simulink model "ADCS_pointing_test"  (R2025b)
settings: Solver=VariableStepAuto  StartTime=0.0  StopTime=t0  FixedStep=0.1  MaxStep=0.1  RelTol=1e-3
values from neighbouring files (symbols this model uses):
  h0 = [1 1 1]*0.5    [parameters.m]
  kd_point = 20    [parameters.m]
  kp_point = 2    [parameters.m]
  omega_0 = [0 0 0.0011]    [parameters.m]
  P = satellite_params()    [individual_test_with_dynamics.m]    (also in parameters.m; test.m = thrusters(:, 1:3))
  q0 = [sqrt(0.5) -sqrt(0.5) 0 0]    [parameters.m]
  ts = 0.1    [parameters.m]
libraries: matrix_library x3, sim3dlib x2, aerolibutil x2
settings Model: Creator=ADMIN  LastModifiedBy=ADMIN
settings DataIOCC: ExternalInput=ds  LoadExternalInput=on

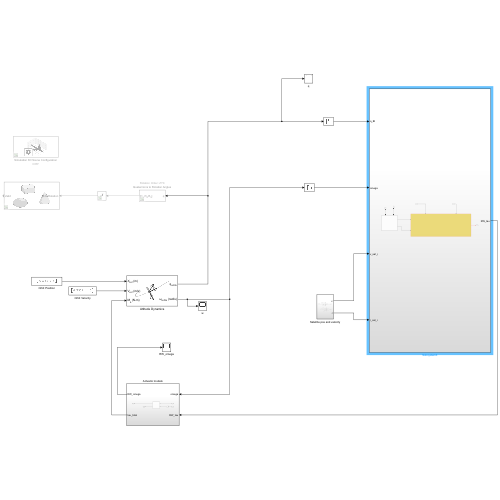
[thumbnail: Simulink's stored preview of the top-level diagram]
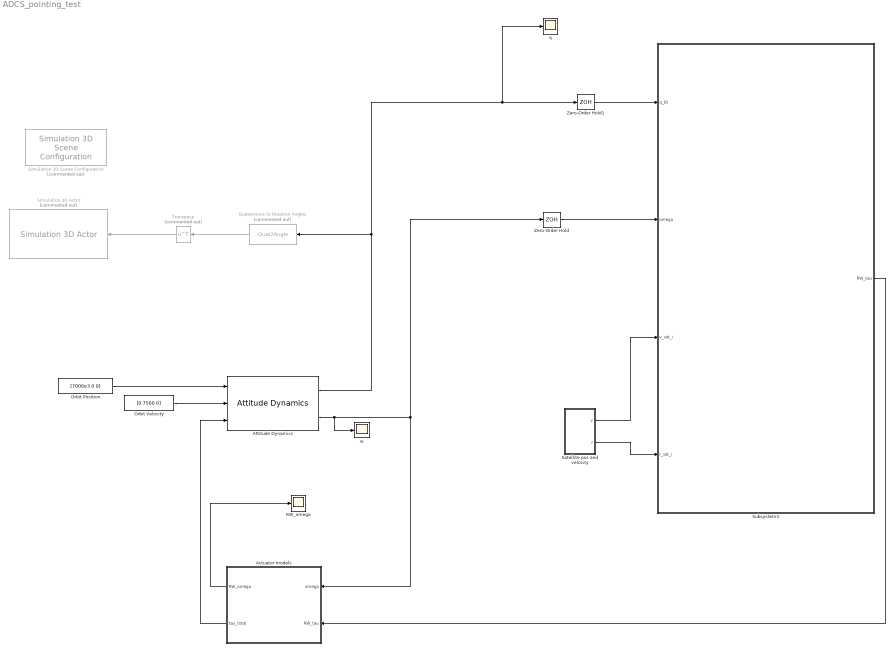
== system ADCS_pointing_test ==
  Actuator models : Subsystem
  Attitude Dynamics : AttitudeDynamics  dateOut=off  mass=P.mass0  inertia=P.I0  outputFuelStatus=off  attitude=q0.'  attitudeRate=omega_0.'  useGravGrad=off  angleUnits=Radians
  Orbit Position : Constant  Value=[7000e3 0 0]
  Orbit Velocity : Constant  Value=[0 7500 0]
  Quaternions to Rotation Angles : Quat2Angle  Commented=on
      settings: AttributesFormatString=Rotation Order: %<rotationOrder>
  RW_omega : Scope
      settings: ActiveDisplayYMinimum=-1.8375  ActiveDisplayYMaximum=1.8375  DataLoggingVariableName=ScopeData5
  Satellite pos and velocity : Subsystem
  Simulation 3D Actor : sim3dlib/Simulation 3D Actor  Priority=1  Commented=on  ActorName=M4V  ParentName=Scene Origin  Operation=Create at setup  InitScriptText=|  SampleTime=-1  Translation=[0 0 0]  Rotation=[0 0 0]  Scale=[1 1 1]*0.1  InputsText=M4V.Rotation  aMode=5  ActorTag=M4V  ActorType=Sim3dActor  ID=C
      | % Reserved keywords:
      | % - Actor : handle to this actor object
      | % - World : handle to the world object
      | 
      | % Examples:
      | 
      | % Create a primitive geometry (optional)
      | % createShape(Actor, 'box', [1 1 1]);
      | 
      | % Initialize values (optional)
      | % Actor.Physics = true;
      | % Actor.Color = [1 0 0];
      | M4V.Mobility = sim3d.utils.MobilityTypes.Movable;
      | 
      | % For simple motion without gravity
      | M4V.Physics = true;
      | M4V.Gravity = false;
      | M4V.Collisions = false;
  Simulation 3D Scene Configuration : sim3dlib/Simulation 3D Scene Configuration  Priority=0  Commented=on  ProjectFormat=Default Scenes  SceneDesc=Space  ProjectName=C:\Program Files\MATLAB\R2025b\toolbox\shared\sim3d_projects\automotive_project_windows\UE\WindowsNoEditor\VehicleSimulation.exe  ScenePath=/Game/Maps/HwStrght  EnableOpenDRIVE=off  vehTagList={'Custom';'M4V';'Scene Origin'}  vehTag=Custom  AttachedCameraRelativeTranslation=[-20000 0 0]  FreeCameraDefaultInitialTranslation=[-6, 0, 2]  AttachedCameraRelativeRotation=[0 0 0]  FreeCameraDefaultInitialRotation=[0, -15, 0]  ViewpointName=Custom  FreeCameraInitialTranslation=[-1500 0 500]  ViewpointTranslation=[0 0 0]  FreeCameraInitialRotation=[0 0 0]  ViewpointRotation=[0 0 0]  OpVisEn=off  Ts=1  EnableWindow=on  EnableRemoteAccess=off  EnableWeather=off  SunAzimuth=90  SunAltitude=40.0  EnableGeospatialSun=off  Latitude=0  Longitude=0  Date=2023-01-01  Time=10:30:00  GeoTimeZone=-5.0  SunDaylightSaving=off  wind=0  clouds=10  EnableVolumetricClouds=off  CloudCoverage=0  CloudAltitude=6  fog=0  rain=0  RaindropsEffect=off  SnowDensity=0  EnableGeospatial=off  TilesetSource=Earth terrain  UseTrueOrigin=off  OriginHeight=200  OriginLatitude=40.744652  OriginLongitude=-73.988864  MapStyle=Aerial  AdditionalAssetIDs=[]  UseAdvancedSunSky=off  SolarTime=11  TimeZone=-5  Day=21  Month=9  Year=2022  UseDaylightSavingTime=on  DSTStartDay=10  DSTStartMonth=3  DSTEndDay=3  DSTEndMonth=11  DSTSwitchHour=2  sensorTag=MainCamera1  sensorId=1  sensorName=MainCamera1  mountLoc=Origin  offsetFlag=off  tmountOffset=[0, 0, 0]  rmountOffset=[0, 0, 0]  HorizontalResolution=1280  VerticalResolution=720  HorizontalFOV=60  mountPoint=[0 0 0]  mountOrientation=[0 0 0]  aMode=0  ID=1  GeoTrigger=Inactive  ViewNameList={'Custom'}  ViewTranslationList={'[-1500 0 500]'}  ViewRotationList={'[0 0 0]'}
      settings: AttributesFormatString=ICRF  LibrarySourceBlock=aerolibsim3d/Simulation 3D Scene Configuration
  Subsystem3 : Subsystem
  Transpose : Math  Commented=on  Operator=transpose
  Zero-Order Hold : ZeroOrderHold  SampleTime=ts
  Zero-Order Hold1 : ZeroOrderHold  SampleTime=ts
  q : Scope
      settings: ActiveDisplayYMinimum=-1.2475163124751956  ActiveDisplayYMaximum=1.2496817270129896  DataLoggingVariableName=ScopeData2
  w : Scope
      settings: ActiveDisplayYMinimum=-0.031776762100484128  ActiveDisplayYMaximum=0.0395431946397378
  wires:
  Orbit Position/1 -> Attitude Dynamics/1
  Orbit Velocity/1 -> Attitude Dynamics/2
  Subsystem3/1(RW_tau) -> Actuator models/2(RW_tau)
  Actuator models/2(tau_total) -> Attitude Dynamics/3
  Transpose/1 -> Simulation 3D Actor/1
  Quaternions to Rotation Angles/1 -> Transpose/1
  Attitude Dynamics/2 -> w/1, Zero-Order Hold/1, Actuator models/1(omega)
  Actuator models/1(RW_omega) -> RW_omega/1
  Satellite pos and velocity/1(v) -> Subsystem3/3(v_sat_i)
  Satellite pos and velocity/2(r) -> Subsystem3/4(r_sat_i)
  Zero-Order Hold/1 -> Subsystem3/2(omega)
  Zero-Order Hold1/1 -> Subsystem3/1(q_BI)
  Attitude Dynamics/1 -> q/1, Zero-Order Hold1/1, Quaternions to Rotation Angles/1

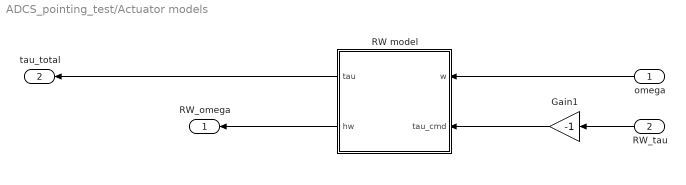
== system ADCS_pointing_test/Actuator models ==
  omega : Inport
  RW_tau : Inport  Port=2
  Gain1 : Gain  Gain=-1
  RW model : Subsystem
  RW_omega : Outport
  tau_total : Outport  Port=2
  wires:
  omega/1 -> RW model/1(w)
  RW_tau/1 -> Gain1/1
  RW model/2(hw) -> RW_omega/1
  RW model/1(tau) -> tau_total/1
  Gain1/1 -> RW model/2(tau_cmd)

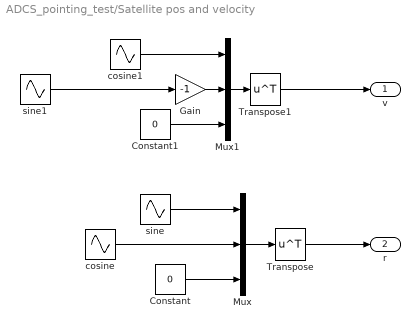
== system ADCS_pointing_test/Satellite pos and velocity ==
  Constant : Constant  Value=0
  Constant1 : Constant  Value=0
  Gain : Gain  Gain=-1
  Mux : Mux  Inputs=3
  Mux1 : Mux  Inputs=3
  Transpose : Math  Operator=transpose
  Transpose1 : Math  Operator=transpose
  cosine : Sin  Amplitude=7e6  Frequency=0.0011  Phase=pi/2  SampleTime=0
  cosine1 : Sin  Amplitude=7e6*0.0011  Frequency=0.0011  Phase=pi/2  SampleTime=0
  sine : Sin  Amplitude=7e6  Frequency=0.0011  SampleTime=0
  sine1 : Sin  Amplitude=7e6*0.0011  Frequency=0.0011  SampleTime=0
  v : Outport
  r : Outport  Port=2
  wires:
  sine/1 -> Mux/1
  cosine1/1 -> Mux1/1
  cosine/1 -> Mux/2
  Gain/1 -> Mux1/2
  Constant/1 -> Mux/3
  Constant1/1 -> Mux1/3
  sine1/1 -> Gain/1
  Mux/1 -> Transpose/1
  Transpose/1 -> r/1
  Mux1/1 -> Transpose1/1
  Transpose1/1 -> v/1

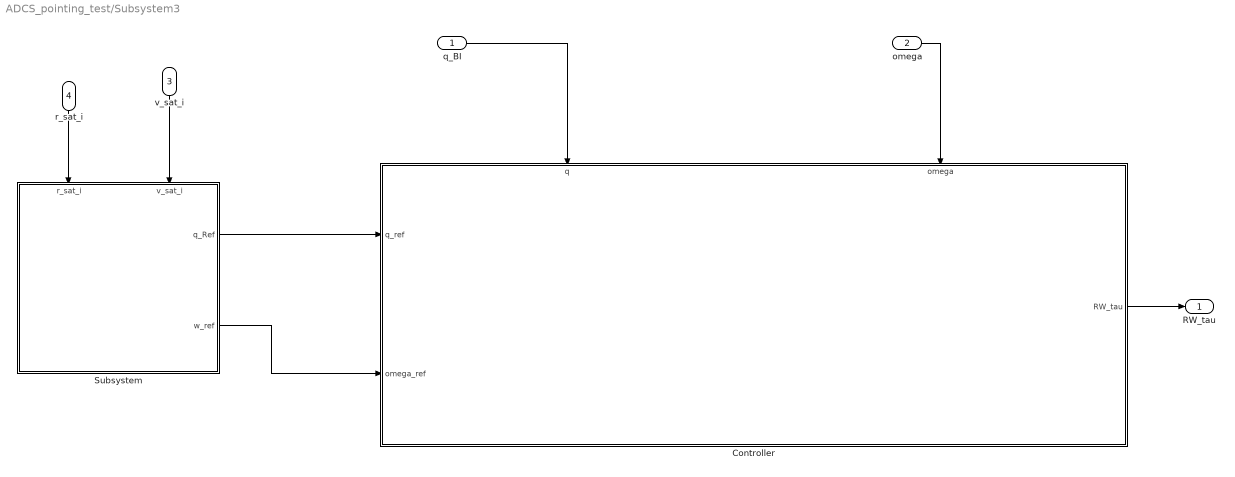
== system ADCS_pointing_test/Subsystem3 ==
  q_BI : Inport
  omega : Inport  Port=2
  v_sat_i : Inport  Port=3
  r_sat_i : Inport  Port=4
  Controller : Subsystem
      settings: PortSchema="{\"entries\":[{\"content\":{\"sides\":[{\"content\":{\"connectorIds\":[\"In1\",\"In2\"]},\"type\":\"ConnectorPlacement.EquallySpacedRectSide\",\"uuid\":\"3d0ce77c-a0dd-4e63-bb58-aa259872b360\"},{\"content\":{\"connectorIds\":[\"Out1\"],\"side\":\"RIGHT\"},\"type\":\"ConnectorPlacement.EquallySpacedRectSide\",\"uuid\":\"c51ce6d0-00d2-499a-9be1-102c03c9909c\"},{\"content\":{\"connectorIds\":[\"In3\",\"In4\"],\"side\":\"TOP\"},\"type\":\"ConnectorPlacement.EquallySpacedRectSide\",\"uuid\":\"ed1e7bc4-2cca-4611-893f-1128994bf2d9\"},{\"content\":{\"side\":\"BOTTOM\"},\"type\":\"ConnectorPlacement.EquallySpacedRectSide\",\"uuid\":\"574e7f6a-1005-4b0c-82f8-22f1ef6841a8\"}]},\"type\":\"ConnectorPlacement.EquallySpacedConnector\",\"uuid\":\"15c446ec-b512-4968-b865-507fd68d8b0b\"}],\"packageUris\":[\"http://schema.mathworks.com/mf0/Connector/R2020b\"],\"version\":\"1.0\"}"
  Subsystem : Subsystem
      settings: PortSchema="{\"entries\":[{\"content\":{\"sides\":[{\"content\":{},\"type\":\"ConnectorPlacement.EquallySpacedRectSide\",\"uuid\":\"74bf1b15-53db-441c-9152-7c9ad8598452\"},{\"content\":{\"connectorIds\":[\"Out1\",\"Out2\"],\"side\":\"RIGHT\"},\"type\":\"ConnectorPlacement.EquallySpacedRectSide\",\"uuid\":\"e98e0885-3f20-4aa1-b3a1-f2c890def05c\"},{\"content\":{\"connectorIds\":[\"In1\",\"In2\"],\"side\":\"TOP\"},\"type\":\"ConnectorPlacement.EquallySpacedRectSide\",\"uuid\":\"f0898a47-7ae2-48e7-af8a-6d6327a5175a\"}]},\"type\":\"ConnectorPlacement.EquallySpacedConnector\",\"uuid\":\"b563a257-d36a-4c1e-a9df-51a9ac9caccd\"}],\"packageUris\":[\"http://schema.mathworks.com/mf0/Connector/R2020b\"],\"version\":\"1.0\"}"
  RW_tau : Outport
  wires:
  Controller/1(RW_tau) -> RW_tau/1
  omega/1 -> Controller/4(omega)
  Subsystem/1(q_Ref) -> Controller/1(q_ref)
  Subsystem/2(w_ref) -> Controller/2(omega_ref)
  v_sat_i/1 -> Subsystem/2(v_sat_i)
  r_sat_i/1 -> Subsystem/1(r_sat_i)
  q_BI/1 -> Controller/3(q)

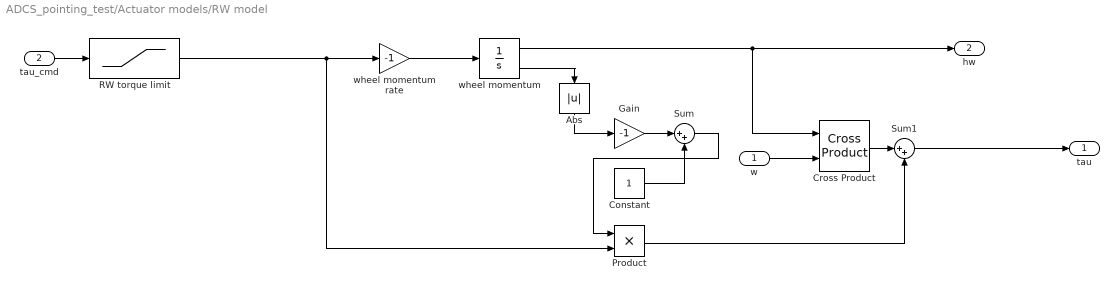
== system ADCS_pointing_test/Actuator models/RW model ==
  w : Inport
  tau_cmd : Inport  Port=2
  Abs : Abs  SaturateOnIntegerOverflow=off
  Constant : Constant
  Cross Product : matrix_library/Cross Product
  Gain : Gain  Gain=-1
  Product : Product
  RW torque limit : Saturate  UpperLimit=P.rw.torque_max  LowerLimit=-P.rw.torque_max
  Sum : Sum  Inputs=|++
  Sum1 : Sum  Inputs=|++
  wheel momentum : Integrator  InitialCondition=h0  LimitOutput=on  UpperSaturationLimit=P.rw.h_max  LowerSaturationLimit=-P.rw.h_max  ShowSaturationPort=on
  wheel momentum rate : Gain  Gain=-1
  tau : Outport
  hw : Outport  Port=2
  wires:
  Abs/1 -> Gain/1
  wheel momentum rate/1 -> wheel momentum/1
  RW torque limit/1 -> Product/2, wheel momentum rate/1
  wheel momentum/1 -> Cross Product/1, hw/1
  wheel momentum/2 -> Abs/1
  Gain/1 -> Sum/1
  Constant/1 -> Sum/2
  Sum/1 -> Product/1
  tau_cmd/1 -> RW torque limit/1
  Product/1 -> Sum1/2
  w/1 -> Cross Product/2
  Cross Product/1 -> Sum1/1
  Sum1/1 -> tau/1

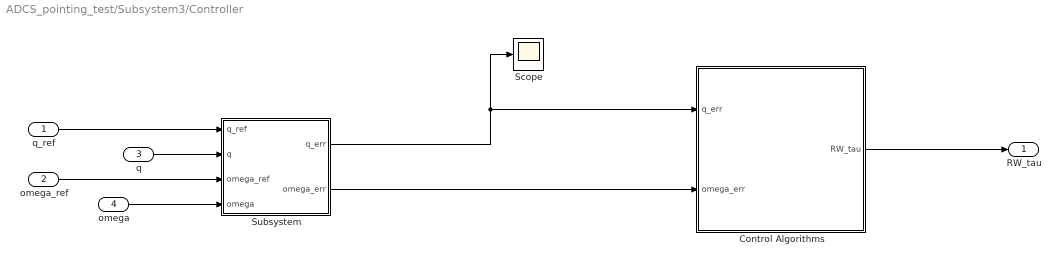
== system ADCS_pointing_test/Subsystem3/Controller ==
  q_ref : Inport
  omega_ref : Inport  Port=2
  q : Inport  Port=3
  omega : Inport  Port=4
  Control Algorithms : Subsystem
  Scope : Scope
      settings: ActiveDisplayYMinimum=-0.87716911871938286  ActiveDisplayYMaximum=0.90484136851718544  DataLoggingVariableName=ScopeData8
  Subsystem : Subsystem
  RW_tau : Outport
  wires:
  Subsystem/1(q_err) -> Scope/1, Control Algorithms/1(q_err)
  Subsystem/2(omega_err) -> Control Algorithms/2(omega_err)
  Control Algorithms/1(RW_tau) -> RW_tau/1
  q_ref/1 -> Subsystem/1(q_ref)
  q/1 -> Subsystem/2(q)
  omega_ref/1 -> Subsystem/3(omega_ref)
  omega/1 -> Subsystem/4(omega)

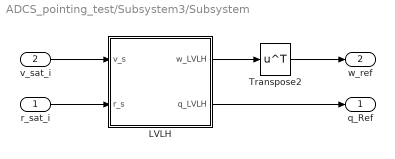
== system ADCS_pointing_test/Subsystem3/Subsystem ==
  r_sat_i : Inport
  v_sat_i : Inport  Port=2
  LVLH : Subsystem
  Transpose2 : Math  Operator=transpose
  q_Ref : Outport
  w_ref : Outport  Port=2
  wires:
  LVLH/1(w_LVLH) -> Transpose2/1
  v_sat_i/1 -> LVLH/1(v_s)
  r_sat_i/1 -> LVLH/2(r_s)
  LVLH/2(q_LVLH) -> q_Ref/1
  Transpose2/1 -> w_ref/1

== system ADCS_pointing_test/Subsystem3/Controller/Control Algorithms ==
  q_err : Inport
  omega_err : Inport  Port=2
  RW Torque Commands : Subsystem
      settings: PortSchema="{\"entries\":[{\"content\":{\"sides\":[{\"content\":{},\"type\":\"ConnectorPlacement.EquallySpacedRectSide\",\"uuid\":\"3d0ce77c-a0dd-4e63-bb58-aa259872b360\"},{\"content\":{\"connectorIds\":[\"Out1\"],\"side\":\"RIGHT\"},\"type\":\"ConnectorPlacement.EquallySpacedRectSide\",\"uuid\":\"c51ce6d0-00d2-499a-9be1-102c03c9909c\"},{\"content\":{\"connectorIds\":[\"In1\",\"In2\"],\"side\":\"TOP\"},\"type\":\"ConnectorPlacement.EquallySpacedRectSide\",\"uuid\":\"ed1e7bc4-2cca-4611-893f-1128994bf2d9\"}]},\"type\":\"ConnectorPlacement.EquallySpacedConnector\",\"uuid\":\"15c446ec-b512-4968-b865-507fd68d8b0b\"}],\"packageUris\":[\"http://schema.mathworks.com/mf0/Connector/R2020b\"],\"version\":\"1.0\"}"
  RW_tau : Outport
  wires:
  omega_err/1 -> RW Torque Commands/1(omega_err)
  q_err/1 -> RW Torque Commands/2(q_err)
  RW Torque Commands/1(tau_cmd) -> RW_tau/1

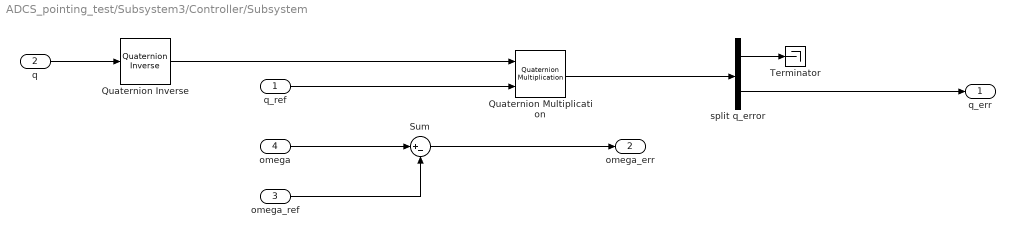
== system ADCS_pointing_test/Subsystem3/Controller/Subsystem ==
  q_ref : Inport
  q : Inport  Port=2
  omega_ref : Inport  Port=3
  omega : Inport  Port=4
  Quaternion Inverse : aerolibutil/Quaternion Inverse
  Quaternion Multiplication : aerolibutil/Quaternion Multiplication
  Sum : Sum  Inputs=|+-
  Terminator : Terminator
  split q_error : Demux  Outputs=[1 3]
  q_err : Outport
  omega_err : Outport  Port=2
  wires:
  q/1 -> Quaternion Inverse/1
  Sum/1 -> omega_err/1
  q_ref/1 -> Quaternion Multiplication/2
  Quaternion Inverse/1 -> Quaternion Multiplication/1
  omega/1 -> Sum/1
  omega_ref/1 -> Sum/2
  split q_error/2 -> q_err/1
  split q_error/1 -> Terminator/1
  Quaternion Multiplication/1 -> split q_error/1

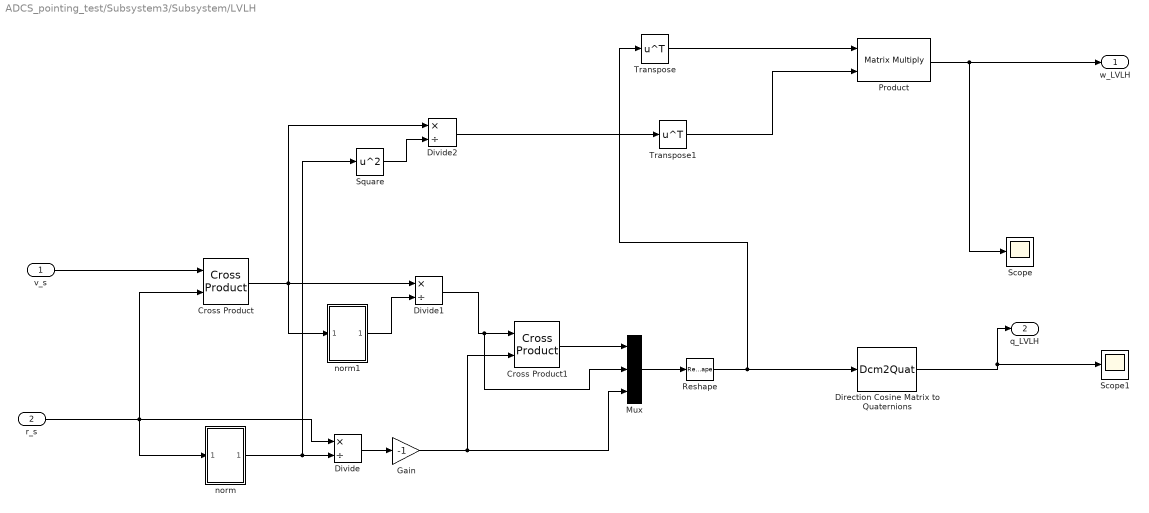
== system ADCS_pointing_test/Subsystem3/Subsystem/LVLH ==
  v_s : Inport
  r_s : Inport  Port=2
  Cross Product : matrix_library/Cross Product
  Cross Product1 : matrix_library/Cross Product
  Direction Cosine Matrix to Quaternions : Dcm2Quat
  Divide : Product  Inputs=*/
  Divide1 : Product  Inputs=*/
  Divide2 : Product  Inputs=*/
  Gain : Gain  Gain=-1
  Mux : Mux  Inputs=3
  Product : Product  Multiplication=Matrix(*)
  Reshape : Reshape  OutputDimensionality=Customize  OutputDimensions=[3,3]
  Scope : Scope
      settings: ActiveDisplayYMinimum=-1  ActiveDisplayYMaximum=1  DataLoggingVariableName=ScopeData4
  Scope1 : Scope
      settings: ActiveDisplayYMinimum=-0.82867069291103368  ActiveDisplayYMaximum=0.87774872275294546
  Square : Math  Operator=square
  Transpose : Math  Operator=transpose
  Transpose1 : Math  Operator=transpose
  norm : Subsystem
  norm1 : Subsystem
  w_LVLH : Outport
  q_LVLH : Outport  Port=2
  wires:
  norm1/1(Out1) -> Divide1/2
  Mux/1 -> Reshape/1
  r_s/1 -> norm/1(In1), Divide/1, Cross Product/2
  v_s/1 -> Cross Product/1
  norm/1(Out1) -> Square/1, Divide/2
  Divide/1 -> Gain/1
  Cross Product/1 -> Divide2/1, Divide1/1, norm1/1(In1)
  Square/1 -> Divide2/2
  Transpose/1 -> Product/1
  Divide2/1 -> Transpose1/1
  Product/1 -> Scope/1, w_LVLH/1
  Cross Product1/1 -> Mux/1
  Divide1/1 -> Mux/2, Cross Product1/1
  Gain/1 -> Mux/3, Cross Product1/2
  Transpose1/1 -> Product/2
  Reshape/1 -> Transpose/1, Direction Cosine Matrix to Quaternions/1
  Direction Cosine Matrix to Quaternions/1 -> Scope1/1, q_LVLH/1

== system ADCS_pointing_test/Subsystem3/Controller/Control Algorithms/RW Torque Commands ==
  omega_err : Inport
  q_err : Inport  Port=2
  POINT : Subsystem  TreatAsAtomicUnit=on
  tau_cmd : Outport
  wires:
  omega_err/1 -> POINT/2(omega_err)
  q_err/1 -> POINT/1(q_err)
  POINT/1(tau_cmd) -> tau_cmd/1

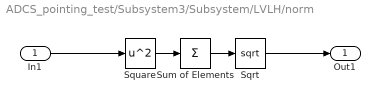
== system ADCS_pointing_test/Subsystem3/Subsystem/LVLH/norm ==
  In1 : Inport
  Sqrt : Sqrt
  Square : Math  Operator=square
  Sum of Elements : Sum  Inputs=+
  Out1 : Outport
  wires:
  In1/1 -> Square/1
  Square/1 -> Sum of Elements/1
  Sum of Elements/1 -> Sqrt/1
  Sqrt/1 -> Out1/1

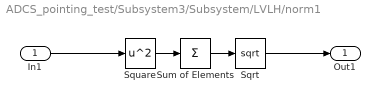
== system ADCS_pointing_test/Subsystem3/Subsystem/LVLH/norm1 ==
  In1 : Inport
  Sqrt : Sqrt
  Square : Math  Operator=square
  Sum of Elements : Sum  Inputs=+
  Out1 : Outport
  wires:
  Sqrt/1 -> Out1/1
  Sum of Elements/1 -> Sqrt/1
  Square/1 -> Sum of Elements/1
  In1/1 -> Square/1

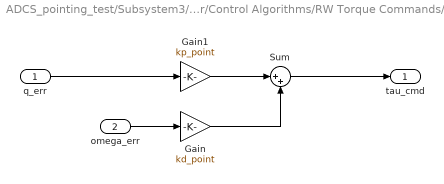
== system ADCS_pointing_test/Subsystem3/Controller/Control Algorithms/RW Torque Commands/POINT ==
  q_err : Inport
  omega_err : Inport  Port=2
  Gain : Gain  Gain=kd_point
  Gain1 : Gain  Gain=kp_point
  Sum : Sum  Inputs=|++
  tau_cmd : Outport
  wires:
  Sum/1 -> tau_cmd/1
  omega_err/1 -> Gain/1
  Gain1/1 -> Sum/1
  Gain/1 -> Sum/2
  q_err/1 -> Gain1/1
